simulink model "model"  (R2025b)
settings: Solver=ode15s  StartTime=0.0  StopTime=900  MaxStep=1e5  RelTol=1e5
values from neighbouring files (symbols this model uses):
  A = [-3 1 ... (first row only)    [init.m]
  A0 = [-sqrt(0.32)  1 ... (first row only)    [init.m]
  B = [1; 9]    [init.m]
  C = [1 0]    [init.m]
  C_xi = [1 0 0 0 0 0 0 0 ... (first row only)    [init.m]
  e_U0 = [0;1]    [init.m]
  e_U1 = [1; 0]    [init.m]
  e_Y0 = [0;1]    [init.m]
  e_Y1 = [1;0]    [init.m]
  gamma = 500    [init.m]
  I = eye(2)    [init.m]
  teta = [0.16 - 2; sqrt(0.32) - 3; 9; 1]    [init.m]
  v0 = [0;0]    [init.m]
settings Model: Creator=eva  LastModifiedBy=eva

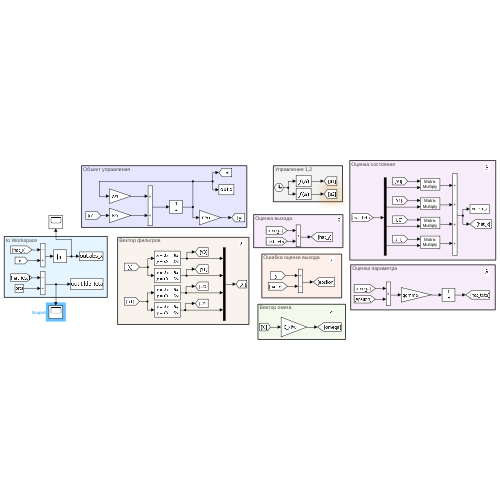
[thumbnail: Simulink's stored preview of the top-level diagram]
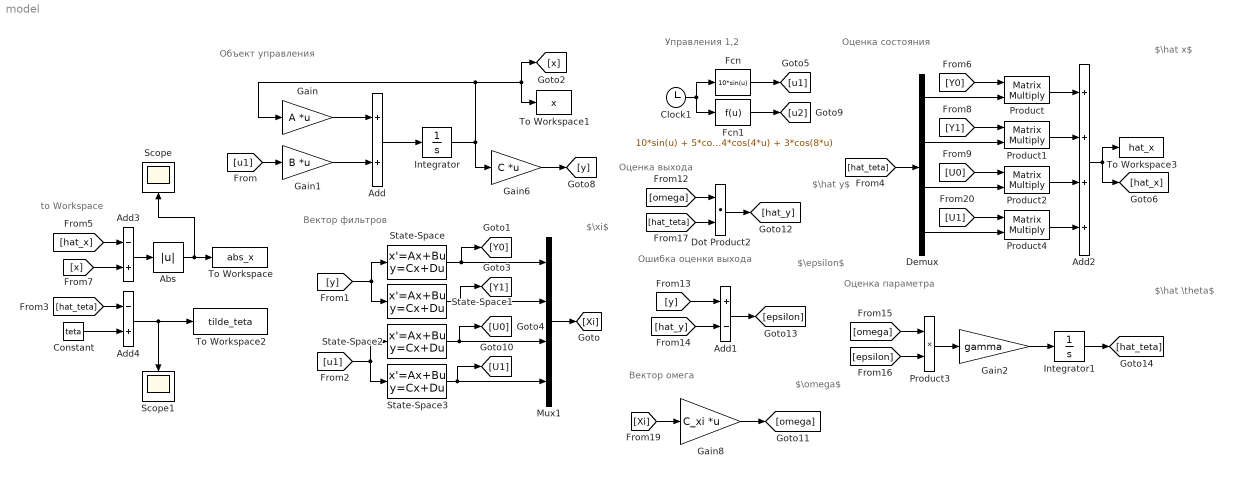
== system model ==
  note: Вектор омега
  note: Ошибка оценки выхода
  note: Оценка выхода
  note: Оценка параметра
  note: $\hat x$
  note: Оценка состояния
  note: $\xi$
  note: Вектор фильтров
  note: to Workspace
  note: Управления 1,2
  note: Объект управления
  note: $\hat \theta$
  note: $\hat y$
  note: $\epsilon$
  note: $\omega$
  Abs : Abs  SaturateOnIntegerOverflow=off
  Add : Sum
  Add1 : Sum  Inputs=+-
  Add2 : Sum  Inputs=++++
  Add3 : Sum  Inputs=-+
  Add4 : Sum  Inputs=-+
  Clock1 : Clock
  Constant : Constant  Value=teta
  Demux : Demux
  Dot Product2 : DotProduct  OutDataTypeStr=Inherit: Inherit via internal rule
  Fcn : Fcn  Expr=10*sin(u)
  Fcn1 : Fcn  Expr=10*sin(u) + 5*cos(2*u) + 4*cos(4*u) + 3*cos(8*u)
  Gain : Gain  Gain=A  Multiplication=Matrix(K*u)
  Gain1 : Gain  Gain=B  Multiplication=Matrix(K*u)
  Gain2 : Gain  Gain=gamma
  Gain6 : Gain  Gain=C  Multiplication=Matrix(K*u)
  Gain8 : Gain  Gain=C_xi  Multiplication=Matrix(K*u)
  Integrator : Integrator  InitialCondition=[0; 0]
  Integrator1 : Integrator  InitialCondition=[0;0;0;0]
  Mux1 : Mux
  Product{,1..2,4} (4 alike) : Product  Multiplication=Matrix(*)
  Product3 : Product
  Scope : Scope
      settings: ActiveDisplayYMinimum=-5  ActiveDisplayYMaximum=95
  Scope1 : Scope
      settings: ActiveDisplayYMinimum=-4
  State-Space : StateSpace  A=A0  B=e_Y0  C=I  D=v0  InitialCondition=[0; 0]
  State-Space1 : StateSpace  A=A0  B=e_Y1  C=I  D=v0  InitialCondition=[0; 0]
  State-Space2 : StateSpace  A=A0  B=e_U0  C=I  D=v0  InitialCondition=[0; 0]
  State-Space3 : StateSpace  A=A0  B=e_U1  C=I  D=v0  InitialCondition=[0; 0]
  To Workspace : ToWorkspace  VariableName=abs_x  SaveFormat=Structure With Time  SampleTime=-1
  To Workspace1 : ToWorkspace  VariableName=x  SaveFormat=Structure With Time  SampleTime=-1
  To Workspace2 : ToWorkspace  VariableName=tilde_teta  SaveFormat=Structure With Time  SampleTime=-1
  To Workspace3 : ToWorkspace  VariableName=hat_x  SaveFormat=Structure With Time  SampleTime=-1
  wires:
  [u1] -> Gain1/1
  Gain/1 -> Add/1
  Add/1 -> Integrator/1
  Gain1/1 -> Add/2
  Integrator/1 -> Gain6/1, To Workspace1/1, [x], Gain/1
  Gain6/1 -> [y]
  [y] -> State-Space1/1, State-Space/1
  State-Space/1 -> Mux1/1, [Y0]
  State-Space1/1 -> Mux1/2, [Y1]
  Fcn1/1 -> [u2]
  State-Space2/1 -> Mux1/3, [U0]
  [omega] -> Dot Product2/1
  [hat_teta] -> Dot Product2/2
  Dot Product2/1 -> [hat_y]
  [y] -> Add1/1
  [hat_y] -> Add1/2
  Add1/1 -> [epsilon]
  Product3/1 -> Gain2/1
  [epsilon] -> Product3/2
  [omega] -> Product3/1
  Gain2/1 -> Integrator1/1
  Integrator1/1 -> [hat_teta]
  Fcn/1 -> [u1]
  [hat_teta] -> Demux/1
  [Y0] -> Product/1
  [Y1] -> Product1/1
  [U0] -> Product2/1
  Product/1 -> Add2/1
  Product1/1 -> Add2/2
  Product2/1 -> Add2/3
  Add2/1 -> To Workspace3/1, [hat_x]
  [hat_x] -> Add3/1
  [x] -> Add3/2
  Add3/1 -> Abs/1
  Clock1/1 -> Fcn/1, Fcn1/1
  State-Space3/1 -> Mux1/4, [U1]
  [U1] -> Product4/1
  Product4/1 -> Add2/4
  Abs/1 -> Scope/1, To Workspace/1
  Constant/1 -> Add4/2
  [hat_teta] -> Add4/1
  [u1] -> State-Space3/1, State-Space2/1
  Mux1/1 -> [Xi]
  [Xi] -> Gain8/1
  Gain8/1 -> [omega]
  Demux/1 -> Product/2
  Demux/2 -> Product1/2
  Demux/3 -> Product2/2
  Demux/4 -> Product4/2
  Add4/1 -> Scope1/1, To Workspace2/1
